simulink model "propellant_consuption"  (R2026a)
settings: Solver=VariableStepAuto
settings Model: Creator=giuse  LastModifiedBy=giuse

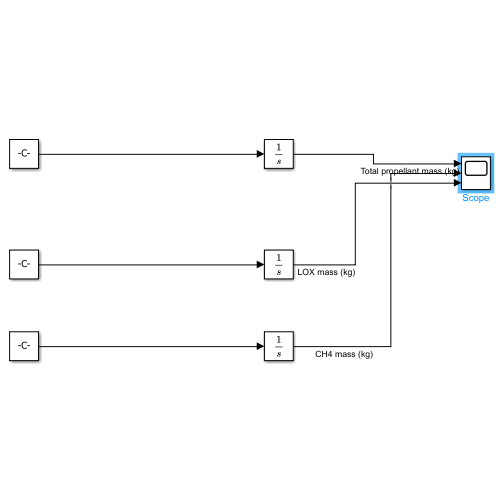
[thumbnail: Simulink's stored preview of the top-level diagram]
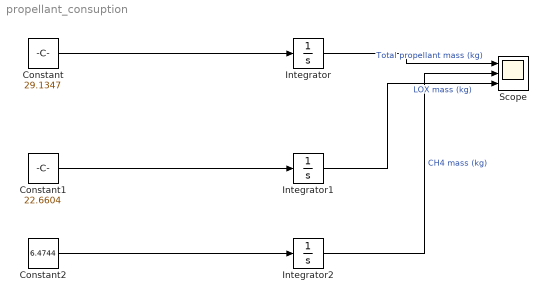
== system propellant_consuption ==
  Constant : Constant  Value=29.1347
  Constant1 : Constant  Value=22.6604
  Constant2 : Constant  Value=6.4744
  Integrator : Integrator
  Integrator1 : Integrator
  Integrator2 : Integrator
  Scope : Scope  NumInputPorts=3
      settings: ActiveDisplayYMinimum=-177.16680012685163  ActiveDisplayYMaximum=485.79128943571857
  wires:
  Constant/1 -> Integrator/1
  Integrator/1 -> Scope/1  "Total propellant mass (kg)"
  Constant1/1 -> Integrator1/1
  Constant2/1 -> Integrator2/1
  Integrator1/1 -> Scope/3  "LOX mass (kg)"
  Integrator2/1 -> Scope/2  "CH4 mass (kg)"
